simulink model "afe_rst_inv_psm_distributed_control_two_delays"  (R2026a)
settings: Solver=ode1be  StopTime=simlength  FixedStep=tc  MaxStep=Tc
values from neighbouring files (symbols this model uses):
  Amplitude_U = 1.16    [grid_fault_generator.m]
  Amplitude_V = Amplitude_U    (= 1.16)    [grid_fault_generator.m]
  Amplitude_W = Amplitude_U    (= 1.16)    [grid_fault_generator.m]
  end_time_LVRT = start_time_LVRT + error_length    [grid_fault_generator.m]
  Igrid_phase_normalization_factor = 270*sqrt(2)    [grid_emulator.m]
  omega_grid_emulator_nom = w_grid    (= 314.159265359)    [grid_emulator.m]
  omega_grid_nom = w_grid    (= 314.159265359)    [grid_emulator.m]
  t_ramp = 20e-3    (= 0.02)    [grid_fault_generator.m]
  ugrid_factor = 1    [grid_emulator.m]
  V_phase_normalization_factor = Vgrid_phase_normalization_factor    [grid_emulator.m]
  Vdc_bez = 1070    [grid_emulator.m]
  Vemu_ref_norm = Vemu_ref * sqrt(2) / V_phase_normalization_factor    [grid_emulator.m]
  vn_eta_pu = 0    [grid_emulator.m]
  vn_xi_pu = 0    [grid_emulator.m]
  vp_xi_pu = 1    [grid_emulator.m]
undefined symbols (not defined in the file or in its folder): Adrso, Aresd, Bresd, CFi, CFu, Cresd, Crso, CTRPIFF_CLIP_RELEASE, dead_time_INV, emf_fb_p, emf_fb_p_ccaller_1, emf_fb_p_ccaller_2, emf_p, emf_p_ccaller_1, emf_p_ccaller_2, fPWM_INV, g0_161Hz, g0_500Hz, g1_161Hz, g1_500Hz, i_grid_neg_eta_lim, i_grid_neg_eta_red_lim, i_grid_neg_xi_lim, i_grid_neg_xi_red_lim, i_grid_pos_eta_lim, i_grid_pos_eta_red_lim, ibez, id_lim, ieta_neg_ref_lim, ieta_pos_ref_lim, iq_lim, ixi_pos_ref_lim, Jm_norm, k_frt_ref, kg, ki_afe, ki_i, ki_id, ki_iq, ki_rc_neg_grid, ki_rc_pos_grid, ki_vs, ki_w, kp_afe, kp_i, kp_id, kp_iq, kp_rc_neg_grid, kp_rc_pos_grid, kp_vs, kp_w, kw, l1, l2, Lalpha_norm, Ld_norm, Ldrso, Lq_norm, Ls_norm, luenberger_l1 ... (+30)
libraries: fl_lib x146, nesl_utility x62, simulink x8, cstblocks_lti x7, sl_discontinuities x3, single_phase_transformer_lib x3, flexshaft_lib x1, permanent_magnet_synchronous_machine x1
(part 8 of 14)

== system afe_rst_inv_psm_distributed_control_two_delays/AFE-Modular/afe_leg_b/driver_board_b/dq_pll/pll_stageB ==
  u_grid_pos_xi : Inport
  u_grid_pos_eta : Inport  Port=2
  -2<x<2 : Saturate  UpperLimit=2  LowerLimit=-2
  Constant4 : Constant  Value=omega_grid_nom
  Product1 : Product  RndMeth=Zero
  Product2 : Product  RndMeth=Zero
  Sum3 : Sum  SaturateOnIntegerOverflow=on
  Sum4 : Sum  SaturateOnIntegerOverflow=on
  Sum5 : Sum  Inputs=++|
  Unit Delay{1..4} (4 alike) : UnitDelay  SampleTime=ts_afe
  bounder1 : MATLAB Function  TreatAsAtomicUnit=on  SystemSampleTime=ts_afe
  kp : Gain  Gain=pll_i1*ts_afe  SaturateOnIntegerOverflow=on  OutDataTypeStr=Inherit: Same as input  ParamDataTypeStr=Inherit: Same as input
  kp1 : Gain  Gain=pll_p  SaturateOnIntegerOverflow=on  OutDataTypeStr=Inherit: Same as input  ParamDataTypeStr=Inherit: Same as input
  kp2 : Gain  Gain=ts_afe  SaturateOnIntegerOverflow=on  OutDataTypeStr=Inherit: Same as input  ParamDataTypeStr=Inherit: Same as input
  gamma_grid_pll : Outport  VectorParamsAs1DForOutWhenUnconnected=off
  wires:
  Unit Delay4/1 -> Sum5/2, Sum3/2
  Sum3/1 -> -2<x<2/1
  Sum4/1 -> bounder1/1(u)
  Unit Delay1/1 -> Sum4/2
  -2<x<2/1 -> Unit Delay4/1  "i1"
  kp2/1 -> Sum4/1
  Constant4/1 -> Product2/2
  [ugrid_unorm_phase_b] -> Unit Delay2/1
  kp/1 -> Sum3/1
  Sum5/1 -> Product2/1
  u_grid_pos_eta/1 -> Unit Delay3/1
  Product2/1 -> kp2/1
  Product1/1 -> kp/1, kp1/1  "V l"
  kp1/1 -> Sum5/1
  bounder1/1(y) -> gamma_grid_pll/1, Unit Delay1/1
  Unit Delay2/1 -> Product1/2
  Unit Delay3/1 -> Product1/1

== system afe_rst_inv_psm_distributed_control_two_delays/AFE-Modular/afe_leg_b/driver_board_b/voltage-current-acquisition/is_eta_neg_ref_fieldbus ==
  is : Inport
  Unit Delay : UnitDelay  SampleTime=ts_afe
  Unit Delay1 : UnitDelay  SampleTime=ts_afe
  Zero-Order Hold : ZeroOrderHold  SampleTime=ts_afe
  is_fb : Outport
  wires:
  is/1 -> Zero-Order Hold/1
  Unit Delay/1 -> Unit Delay1/1
  Zero-Order Hold/1 -> Unit Delay/1
  Unit Delay1/1 -> is_fb/1

== system afe_rst_inv_psm_distributed_control_two_delays/AFE-Modular/afe_leg_b/driver_board_b/voltage-current-acquisition/is_eta_pos_ref_fieldbus ==
  is : Inport
  Unit Delay : UnitDelay  SampleTime=ts_afe
  Unit Delay1 : UnitDelay  SampleTime=ts_afe
  Zero-Order Hold : ZeroOrderHold  SampleTime=ts_afe
  is_fb : Outport
  wires:
  is/1 -> Zero-Order Hold/1
  Unit Delay/1 -> Unit Delay1/1
  Zero-Order Hold/1 -> Unit Delay/1
  Unit Delay1/1 -> is_fb/1

== system afe_rst_inv_psm_distributed_control_two_delays/AFE-Modular/afe_leg_b/driver_board_b/voltage-current-acquisition/is_xi_neg_ref_fieldbus ==
  is : Inport
  Unit Delay : UnitDelay  SampleTime=ts_afe
  Unit Delay1 : UnitDelay  SampleTime=ts_afe
  Zero-Order Hold : ZeroOrderHold  SampleTime=ts_afe
  is_fb : Outport
  wires:
  is/1 -> Zero-Order Hold/1
  Unit Delay/1 -> Unit Delay1/1
  Zero-Order Hold/1 -> Unit Delay/1
  Unit Delay1/1 -> is_fb/1

== system afe_rst_inv_psm_distributed_control_two_delays/AFE-Modular/afe_leg_b/driver_board_b/voltage-current-acquisition/isa_measure ==
  is : Inport
  Gain : Gain  Gain=1/Igrid_phase_normalization_factor
  Quantizer : Quantizer  QuantizationInterval=CurrentQuantization
  Unit Delay : UnitDelay  SampleTime=ts_afe
  Zero-Order Hold : ZeroOrderHold  SampleTime=ts_afe
  is_pu : Outport
  wires:
  Quantizer/1 -> Zero-Order Hold/1
  Gain/1 -> is_pu/1
  Zero-Order Hold/1 -> Unit Delay/1
  Unit Delay/1 -> Gain/1
  is/1 -> Quantizer/1

== system afe_rst_inv_psm_distributed_control_two_delays/AFE-Modular/afe_leg_b/driver_board_b/voltage-current-acquisition/isb_fieldbus ==
  is : Inport
  Unit Delay : UnitDelay  SampleTime=ts_afe
  Unit Delay1 : UnitDelay  SampleTime=ts_afe
  Zero-Order Hold : ZeroOrderHold  SampleTime=ts_afe
  is_fb : Outport
  wires:
  is/1 -> Zero-Order Hold/1
  Unit Delay/1 -> Unit Delay1/1
  Zero-Order Hold/1 -> Unit Delay/1
  Unit Delay1/1 -> is_fb/1

== system afe_rst_inv_psm_distributed_control_two_delays/AFE-Modular/afe_leg_b/driver_board_b/voltage-current-acquisition/isc_fieldbus ==
  is : Inport
  Unit Delay : UnitDelay  SampleTime=ts_afe
  Unit Delay1 : UnitDelay  SampleTime=ts_afe
  Zero-Order Hold : ZeroOrderHold  SampleTime=ts_afe
  is_fb : Outport
  wires:
  is/1 -> Zero-Order Hold/1
  Unit Delay/1 -> Unit Delay1/1
  Zero-Order Hold/1 -> Unit Delay/1
  Unit Delay1/1 -> is_fb/1

== system afe_rst_inv_psm_distributed_control_two_delays/AFE-Modular/afe_leg_b/driver_board_b/voltage-current-acquisition/ixi_ref_fieldbus ==
  is : Inport
  Unit Delay : UnitDelay  SampleTime=ts_afe
  Unit Delay1 : UnitDelay  SampleTime=ts_afe
  Zero-Order Hold : ZeroOrderHold  SampleTime=ts_afe
  is_fb : Outport
  wires:
  is/1 -> Zero-Order Hold/1
  Unit Delay/1 -> Unit Delay1/1
  Zero-Order Hold/1 -> Unit Delay/1
  Unit Delay1/1 -> is_fb/1

== system afe_rst_inv_psm_distributed_control_two_delays/AFE-Modular/afe_leg_b/driver_board_b/voltage-current-acquisition/ixi_ref_fieldbus1 ==
  is : Inport
  Unit Delay : UnitDelay  SampleTime=ts_afe
  Unit Delay1 : UnitDelay  SampleTime=ts_afe
  Zero-Order Hold : ZeroOrderHold  SampleTime=ts_afe
  is_fb : Outport
  wires:
  is/1 -> Zero-Order Hold/1
  Unit Delay/1 -> Unit Delay1/1
  Zero-Order Hold/1 -> Unit Delay/1
  Unit Delay1/1 -> is_fb/1

== system afe_rst_inv_psm_distributed_control_two_delays/AFE-Modular/afe_leg_b/driver_board_b/voltage-current-acquisition/ub_ctrl_fieldbus ==
  u_ctrl : Inport
  Unit Delay : UnitDelay  SampleTime=ts_afe
  Unit Delay1 : UnitDelay  SampleTime=ts_afe
  Zero-Order Hold : ZeroOrderHold  SampleTime=ts_afe
  u_ctrl_fb : Outport
  wires:
  u_ctrl/1 -> Zero-Order Hold/1
  Unit Delay/1 -> Unit Delay1/1
  Zero-Order Hold/1 -> Unit Delay/1
  Unit Delay1/1 -> u_ctrl_fb/1

== system afe_rst_inv_psm_distributed_control_two_delays/AFE-Modular/afe_leg_b/driver_board_b/voltage-current-acquisition/uc_ctrl_fieldbus ==
  u_ctrl : Inport
  Unit Delay : UnitDelay  SampleTime=ts_afe
  Unit Delay1 : UnitDelay  SampleTime=ts_afe
  Zero-Order Hold : ZeroOrderHold  SampleTime=ts_afe
  u_ctrl_fb : Outport
  wires:
  u_ctrl/1 -> Zero-Order Hold/1
  Unit Delay/1 -> Unit Delay1/1
  Zero-Order Hold/1 -> Unit Delay/1
  Unit Delay1/1 -> u_ctrl_fb/1

== system afe_rst_inv_psm_distributed_control_two_delays/AFE-Modular/afe_leg_b/driver_board_b/voltage-current-acquisition/uga_measure ==
  ug : Inport
  Gain : Gain  Gain=1/V_phase_normalization_factor
  Quantizer : Quantizer  QuantizationInterval=CurrentQuantization
  Unit Delay : UnitDelay  SampleTime=ts_afe
  Zero-Order Hold : ZeroOrderHold  SampleTime=ts_afe
  ug_pu : Outport
  wires:
  ug/1 -> Quantizer/1
  Unit Delay/1 -> Gain/1
  Zero-Order Hold/1 -> Unit Delay/1
  Gain/1 -> ug_pu/1
  Quantizer/1 -> Zero-Order Hold/1

== system afe_rst_inv_psm_distributed_control_two_delays/AFE-Modular/afe_leg_b/driver_board_b/voltage-current-acquisition/ugb_fieldbus ==
  ug : Inport
  Unit Delay : UnitDelay  SampleTime=ts_afe
  Unit Delay1 : UnitDelay  SampleTime=ts_afe
  Zero-Order Hold : ZeroOrderHold  SampleTime=ts_afe
  ug_fb : Outport
  wires:
  ug/1 -> Zero-Order Hold/1
  Unit Delay/1 -> Unit Delay1/1
  Zero-Order Hold/1 -> Unit Delay/1
  Unit Delay1/1 -> ug_fb/1

== system afe_rst_inv_psm_distributed_control_two_delays/AFE-Modular/afe_leg_b/driver_board_b/voltage-current-acquisition/ugc_fieldbus ==
  ug : Inport
  Unit Delay : UnitDelay  SampleTime=ts_afe
  Unit Delay1 : UnitDelay  SampleTime=ts_afe
  Zero-Order Hold : ZeroOrderHold  SampleTime=ts_afe
  ug_fb : Outport
  wires:
  ug/1 -> Zero-Order Hold/1
  Unit Delay/1 -> Unit Delay1/1
  Zero-Order Hold/1 -> Unit Delay/1
  Unit Delay1/1 -> ug_fb/1

== system afe_rst_inv_psm_distributed_control_two_delays/AFE-Modular/afe_leg_b/modulator/sv_pwm/modulator ==
  u : Inport
  v : Inport  Port=2
  w : Inport  Port=3
  Bus Creator : BusCreator  Inputs=6
  PWM generator 1 : Subsystem  mask{f=fPWM_INV, ph=0, m_up=0.98, m_low=0.02, dead_time=dead_time_INV, vg_firing=15, polarity=1}
      mask prompts: f "Frequency"; ph "Phase"; m_up "Max Input Modulation Value"; m_low "Min Input Modulation Value"; dead_time "Dead Time"; vg_firing "Gate Voltage"
  PWM generator 2 : Subsystem  mask{f=fPWM_INV, ph=0, m_up=0.98, m_low=0.02, dead_time=dead_time_INV, vg_firing=15, polarity=1}
      mask prompts: f "Frequency"; ph "Phase"; m_up "Max Input Modulation Value"; m_low "Min Input Modulation Value"; dead_time "Dead Time"; vg_firing "Gate Voltage"
  PWM generator 3 : Subsystem  mask{f=fPWM_INV, ph=0, m_up=0.98, m_low=0.02, dead_time=dead_time_INV, vg_firing=15, polarity=1}
      mask prompts: f "Frequency"; ph "Phase"; m_up "Max Input Modulation Value"; m_low "Min Input Modulation Value"; dead_time "Dead Time"; vg_firing "Gate Voltage"
  firing_gates : Outport
  wires:
  PWM generator 1/1(m1) -> Bus Creator/1  "pwm_u_top"
  PWM generator 3/2(m2) -> Bus Creator/6  "pwm_w_bottom"
  PWM generator 2/2(m2) -> Bus Creator/4  "pwm_v_bottom"
  PWM generator 3/1(m1) -> Bus Creator/5  "pwm_w_top"
  PWM generator 2/1(m1) -> Bus Creator/3  "pwm_v_top"
  Bus Creator/1 -> firing_gates/1
  PWM generator 1/2(m2) -> Bus Creator/2  "pwm_u_bottom"
  v/1 -> PWM generator 2/1(m_index)
  w/1 -> PWM generator 3/1(m_index)
  u/1 -> PWM generator 1/1(m_index)

== system afe_rst_inv_psm_distributed_control_two_delays/AFE-Modular/afe_leg_c/driver_board_c/current_ctrl/phase_current_control ==
  In1 : Inport
  is_abc : Inport  Port=2
  Bus Creator1 : BusCreator  Inputs=2
  Bus Creator2 : BusCreator  Inputs=3
  Bus Selector1 : BusSelector  OutputSignals=usa_ctrl,usb_ctrl,usc_ctrl
  MATLAB Function : MATLAB Function  TreatAsAtomicUnit=on
  Selector : Selector  InputPortWidth=3  IndexOptions=Index vector (dialog)  Indices=3  OutputSizes=1
  Unit Delay2 : UnitDelay  SampleTime=ts_afe
  Unit Delay3 : UnitDelay  SampleTime=ts_afe
  isc_ref/isc : Scope  NumInputPorts=2
      settings: SampleTime=ts_afe  ActiveDisplayYMinimum=-6.6016  ActiveDisplayYMaximum=2.92896
  phase-current-control-dbc : Subsystem
  us_alphabeta_ctrl : Outport  VectorParamsAs1DForOutWhenUnconnected=off
  tag scope: usc_ctrl_dbc=global
  wires:
  Bus Creator1/1 -> us_alphabeta_ctrl/1
  Unit Delay2/1 -> Bus Creator1/1  "us_alpha_ctrl"
  Bus Selector1/1 -> MATLAB Function/1(a)  "<usa_ctrl>"
  MATLAB Function/2(beta) -> Unit Delay3/1
  Bus Selector1/2 -> MATLAB Function/2(b)  "<usb_ctrl>"
  Unit Delay3/1 -> Bus Creator1/2  "us_beta_ctrl"
  MATLAB Function/1(alpha) -> Unit Delay2/1
  Bus Selector1/3 -> MATLAB Function/3(c)  "<usc_ctrl>"
  is_abc/1 -> isc_ref/isc/2, phase-current-control-dbc/2(is_abc)  "isc"
  In1/1 -> Selector/1
  phase-current-control-dbc/1(Out1) -> Bus Creator2/3, [usc_ctrl_dbc]  "usc_ctrl"
  [usb_ctrl_dbb_fb_dbc] -> Bus Creator2/2  "usb_ctrl"
  [usa_ctrl_dba_fb_dbc] -> Bus Creator2/1  "usa_ctrl"
  Bus Creator2/1 -> Bus Selector1/1  "us_abc_ctrl"
  Selector/1 -> isc_ref/isc/1, phase-current-control-dbc/1(In1)  "isc_ref"

== system afe_rst_inv_psm_distributed_control_two_delays/AFE-Modular/afe_leg_c/driver_board_c/current_ctrl/xieta2abc ==
  pos_xi : Inport
  pos_eta : Inport  Port=2
  neg_xi : Inport  Port=3
  neg_eta : Inport  Port=4
  gamma : Inport  Port=5
  MATLAB Function2 : MATLAB Function  TreatAsAtomicUnit=on
  Mux : Mux  Inputs=3
  Negative Sequence : MATLAB Function  TreatAsAtomicUnit=on
  Positive Sequence : MATLAB Function  TreatAsAtomicUnit=on
  Sum : Sum  Inputs=|++
  Sum1 : Sum  Inputs=|++
  i_abc_reference : Outport
  wires:
  Mux/1 -> i_abc_reference/1  "i_abc_reference"
  pos_eta/1 -> Positive Sequence/2(eta)
  pos_xi/1 -> Positive Sequence/1(xi)
  neg_xi/1 -> Negative Sequence/1(xi)
  Sum1/1 -> MATLAB Function2/2(beta)
  MATLAB Function2/2(b) -> Mux/2  "i_b"
  Negative Sequence/2(beta) -> Sum1/2
  Positive Sequence/1(alpha) -> Sum/1
  Negative Sequence/1(alpha) -> Sum/2
  MATLAB Function2/3(c) -> Mux/3  "i_c"
  gamma/1 -> Positive Sequence/3(gamma), Negative Sequence/3(gamma)
  Sum/1 -> MATLAB Function2/1(alpha)
  Positive Sequence/2(beta) -> Sum1/1
  MATLAB Function2/1(a) -> Mux/1  "i_a"
  neg_eta/1 -> Negative Sequence/2(eta)

== system afe_rst_inv_psm_distributed_control_two_delays/AFE-Modular/afe_leg_c/driver_board_c/dq_pll/pll_stageA ==
  gamma_grid : Inport
  Math Function : Math  Operator=magnitude^2  SignedPower=on
  Math Function1 : Math  Operator=magnitude^2  SignedPower=on
  Reciprocal Sqrt : Sqrt  Operator=rSqrt
  Saturation : Saturate  UpperLimit=inf  LowerLimit=0.02
  Sum : Sum  Inputs=|++
  mormalization_and_transformation : Subsystem
  sequences : Subsystem
  u_grid_pos_xi : Outport  VectorParamsAs1DForOutWhenUnconnected=off
  u_grid_pos_eta : Outport  Port=2  VectorParamsAs1DForOutWhenUnconnected=off
  tag scope: ugrid_unorm_phase_c=global
  wires:
  mormalization_and_transformation/1(ug_alpha) -> Math Function/1, sequences/1(u_grid_alpha)
  mormalization_and_transformation/2(ug_beta) -> Math Function1/1, sequences/2(u_grid_beta)
  Math Function/1 -> Sum/1
  Math Function1/1 -> Sum/2
  Sum/1 -> Saturation/1
  Reciprocal Sqrt/1 -> [ugrid_unorm_phase_c]
  Saturation/1 -> Reciprocal Sqrt/1
  gamma_grid/1 -> sequences/3(gamma_grid)
  sequences/1(u_grid_pos_xi) -> u_grid_pos_xi/1
  sequences/2(u_grid_pos_eta) -> u_grid_pos_eta/1
  [ugb_pu_dbb_fb_dbc] -> mormalization_and_transformation/2(ug_b)
  [uga_pu_dba_fb_dbc] -> mormalization_and_transformation/1(ug_a)
  [ugc_pu_dbc] -> mormalization_and_transformation/3(ug_c)

== system afe_rst_inv_psm_distributed_control_two_delays/AFE-Modular/afe_leg_c/driver_board_c/dq_pll/pll_stageB ==
  u_grid_pos_xi : Inport
  u_grid_pos_eta : Inport  Port=2
  -2<x<2 : Saturate  UpperLimit=2  LowerLimit=-2
  Constant4 : Constant  Value=omega_grid_nom
  Product1 : Product  RndMeth=Zero
  Product2 : Product  RndMeth=Zero
  Sum3 : Sum  SaturateOnIntegerOverflow=on
  Sum4 : Sum  SaturateOnIntegerOverflow=on
  Sum5 : Sum  Inputs=++|
  Unit Delay{1..4} (4 alike) : UnitDelay  SampleTime=ts_afe
  bounder1 : MATLAB Function  TreatAsAtomicUnit=on  SystemSampleTime=ts_afe
  kp : Gain  Gain=pll_i1*ts_afe  SaturateOnIntegerOverflow=on  OutDataTypeStr=Inherit: Same as input  ParamDataTypeStr=Inherit: Same as input
  kp1 : Gain  Gain=pll_p  SaturateOnIntegerOverflow=on  OutDataTypeStr=Inherit: Same as input  ParamDataTypeStr=Inherit: Same as input
  kp2 : Gain  Gain=ts_afe  SaturateOnIntegerOverflow=on  OutDataTypeStr=Inherit: Same as input  ParamDataTypeStr=Inherit: Same as input
  gamma_grid_pll : Outport  VectorParamsAs1DForOutWhenUnconnected=off
  wires:
  Unit Delay4/1 -> Sum3/2, Sum5/2
  Sum3/1 -> -2<x<2/1
  Sum4/1 -> bounder1/1(u)
  Unit Delay1/1 -> Sum4/2
  -2<x<2/1 -> Unit Delay4/1  "i1"
  kp2/1 -> Sum4/1
  Constant4/1 -> Product2/2
  [ugrid_unorm_phase_c] -> Unit Delay2/1
  kp/1 -> Sum3/1
  Sum5/1 -> Product2/1
  u_grid_pos_eta/1 -> Unit Delay3/1
  Product2/1 -> kp2/1
  Product1/1 -> kp/1, kp1/1  "V l"
  kp1/1 -> Sum5/1
  bounder1/1(y) -> gamma_grid_pll/1, Unit Delay1/1
  Unit Delay2/1 -> Product1/2
  Unit Delay3/1 -> Product1/1

== system afe_rst_inv_psm_distributed_control_two_delays/AFE-Modular/afe_leg_c/driver_board_c/voltage-current-acquisition/is_eta_neg_ref_fieldbus ==
  is : Inport
  Unit Delay : UnitDelay  SampleTime=ts_afe
  Unit Delay1 : UnitDelay  SampleTime=ts_afe
  Zero-Order Hold : ZeroOrderHold  SampleTime=ts_afe
  is_fb : Outport
  wires:
  is/1 -> Zero-Order Hold/1
  Unit Delay/1 -> Unit Delay1/1
  Zero-Order Hold/1 -> Unit Delay/1
  Unit Delay1/1 -> is_fb/1

== system afe_rst_inv_psm_distributed_control_two_delays/AFE-Modular/afe_leg_c/driver_board_c/voltage-current-acquisition/is_eta_pos_ref_fieldbus ==
  is : Inport
  Unit Delay : UnitDelay  SampleTime=ts_afe
  Unit Delay1 : UnitDelay  SampleTime=ts_afe
  Zero-Order Hold : ZeroOrderHold  SampleTime=ts_afe
  is_fb : Outport
  wires:
  is/1 -> Zero-Order Hold/1
  Unit Delay/1 -> Unit Delay1/1
  Zero-Order Hold/1 -> Unit Delay/1
  Unit Delay1/1 -> is_fb/1

== system afe_rst_inv_psm_distributed_control_two_delays/AFE-Modular/afe_leg_c/driver_board_c/voltage-current-acquisition/is_xi_neg_ref_fieldbus ==
  is : Inport
  Unit Delay : UnitDelay  SampleTime=ts_afe
  Unit Delay1 : UnitDelay  SampleTime=ts_afe
  Zero-Order Hold : ZeroOrderHold  SampleTime=ts_afe
  is_fb : Outport
  wires:
  is/1 -> Zero-Order Hold/1
  Unit Delay/1 -> Unit Delay1/1
  Zero-Order Hold/1 -> Unit Delay/1
  Unit Delay1/1 -> is_fb/1

== system afe_rst_inv_psm_distributed_control_two_delays/AFE-Modular/afe_leg_c/driver_board_c/voltage-current-acquisition/isb_fieldbus ==
  is : Inport
  Unit Delay : UnitDelay  SampleTime=ts_afe
  Unit Delay1 : UnitDelay  SampleTime=ts_afe
  Zero-Order Hold : ZeroOrderHold  SampleTime=ts_afe
  is_fb : Outport
  wires:
  is/1 -> Zero-Order Hold/1
  Unit Delay/1 -> Unit Delay1/1
  Zero-Order Hold/1 -> Unit Delay/1
  Unit Delay1/1 -> is_fb/1

== system afe_rst_inv_psm_distributed_control_two_delays/AFE-Modular/afe_leg_c/driver_board_c/voltage-current-acquisition/isc_fieldbus ==
  is : Inport
  Unit Delay : UnitDelay  SampleTime=ts_afe
  Unit Delay1 : UnitDelay  SampleTime=ts_afe
  Zero-Order Hold : ZeroOrderHold  SampleTime=ts_afe
  is_fb : Outport
  wires:
  is/1 -> Zero-Order Hold/1
  Unit Delay/1 -> Unit Delay1/1
  Zero-Order Hold/1 -> Unit Delay/1
  Unit Delay1/1 -> is_fb/1

== system afe_rst_inv_psm_distributed_control_two_delays/AFE-Modular/afe_leg_c/driver_board_c/voltage-current-acquisition/isc_measure_and_normalization ==
  is : Inport
  Gain : Gain  Gain=1/Igrid_phase_normalization_factor
  Quantizer : Quantizer  QuantizationInterval=CurrentQuantization
  Unit Delay : UnitDelay  SampleTime=ts_afe
  Zero-Order Hold : ZeroOrderHold  SampleTime=ts_afe
  is_pu : Outport
  wires:
  Quantizer/1 -> Zero-Order Hold/1
  Gain/1 -> is_pu/1
  Zero-Order Hold/1 -> Unit Delay/1
  Unit Delay/1 -> Gain/1
  is/1 -> Quantizer/1

== system afe_rst_inv_psm_distributed_control_two_delays/AFE-Modular/afe_leg_c/driver_board_c/voltage-current-acquisition/ixi_ref_fieldbus ==
  is : Inport
  Unit Delay : UnitDelay  SampleTime=ts_afe
  Unit Delay1 : UnitDelay  SampleTime=ts_afe
  Zero-Order Hold : ZeroOrderHold  SampleTime=ts_afe
  is_fb : Outport
  wires:
  is/1 -> Zero-Order Hold/1
  Unit Delay/1 -> Unit Delay1/1
  Zero-Order Hold/1 -> Unit Delay/1
  Unit Delay1/1 -> is_fb/1

== system afe_rst_inv_psm_distributed_control_two_delays/AFE-Modular/afe_leg_c/driver_board_c/voltage-current-acquisition/ixi_ref_fieldbus1 ==
  is : Inport
  Unit Delay : UnitDelay  SampleTime=ts_afe
  Unit Delay1 : UnitDelay  SampleTime=ts_afe
  Zero-Order Hold : ZeroOrderHold  SampleTime=ts_afe
  is_fb : Outport
  wires:
  is/1 -> Zero-Order Hold/1
  Unit Delay/1 -> Unit Delay1/1
  Zero-Order Hold/1 -> Unit Delay/1
  Unit Delay1/1 -> is_fb/1

== system afe_rst_inv_psm_distributed_control_two_delays/AFE-Modular/afe_leg_c/driver_board_c/voltage-current-acquisition/ub_ctrl_fieldbus ==
  u_ctrl : Inport
  Unit Delay : UnitDelay  SampleTime=ts_afe
  Unit Delay1 : UnitDelay  SampleTime=ts_afe
  Zero-Order Hold : ZeroOrderHold  SampleTime=ts_afe
  u_ctrl_fb : Outport
  wires:
  u_ctrl/1 -> Zero-Order Hold/1
  Unit Delay/1 -> Unit Delay1/1
  Zero-Order Hold/1 -> Unit Delay/1
  Unit Delay1/1 -> u_ctrl_fb/1

== system afe_rst_inv_psm_distributed_control_two_delays/AFE-Modular/afe_leg_c/driver_board_c/voltage-current-acquisition/uc_ctrl_fieldbus ==
  u_ctrl : Inport
  Unit Delay : UnitDelay  SampleTime=ts_afe
  Unit Delay1 : UnitDelay  SampleTime=ts_afe
  Zero-Order Hold : ZeroOrderHold  SampleTime=ts_afe
  u_ctrl_fb : Outport
  wires:
  u_ctrl/1 -> Zero-Order Hold/1
  Unit Delay/1 -> Unit Delay1/1
  Zero-Order Hold/1 -> Unit Delay/1
  Unit Delay1/1 -> u_ctrl_fb/1

== system afe_rst_inv_psm_distributed_control_two_delays/AFE-Modular/afe_leg_c/driver_board_c/voltage-current-acquisition/uga_fieldbus ==
  ug : Inport
  Unit Delay : UnitDelay  SampleTime=ts_afe
  Unit Delay1 : UnitDelay  SampleTime=ts_afe
  Zero-Order Hold : ZeroOrderHold  SampleTime=ts_afe
  ug_fb : Outport
  wires:
  ug/1 -> Zero-Order Hold/1
  Zero-Order Hold/1 -> Unit Delay/1
  Unit Delay/1 -> Unit Delay1/1
  Unit Delay1/1 -> ug_fb/1

== system afe_rst_inv_psm_distributed_control_two_delays/AFE-Modular/afe_leg_c/driver_board_c/voltage-current-acquisition/ugb_fieldbus ==
  ug : Inport
  Unit Delay : UnitDelay  SampleTime=ts_afe
  Unit Delay1 : UnitDelay  SampleTime=ts_afe
  Zero-Order Hold : ZeroOrderHold  SampleTime=ts_afe
  ug_fb : Outport
  wires:
  ug/1 -> Zero-Order Hold/1
  Unit Delay/1 -> Unit Delay1/1
  Zero-Order Hold/1 -> Unit Delay/1
  Unit Delay1/1 -> ug_fb/1

== system afe_rst_inv_psm_distributed_control_two_delays/AFE-Modular/afe_leg_c/driver_board_c/voltage-current-acquisition/ugc_measure_and_normalization ==
  ug : Inport
  Gain : Gain  Gain=1/V_phase_normalization_factor
  Quantizer : Quantizer  QuantizationInterval=CurrentQuantization
  Unit Delay : UnitDelay  SampleTime=ts_afe
  Zero-Order Hold : ZeroOrderHold  SampleTime=ts_afe
  ug_pu : Outport
  wires:
  ug/1 -> Quantizer/1
  Unit Delay/1 -> Gain/1
  Zero-Order Hold/1 -> Unit Delay/1
  Gain/1 -> ug_pu/1
  Quantizer/1 -> Zero-Order Hold/1

== system afe_rst_inv_psm_distributed_control_two_delays/AFE-Modular/afe_leg_c/modulator/sv_pwm/modulator ==
  u : Inport
  v : Inport  Port=2
  w : Inport  Port=3
  Bus Creator : BusCreator  Inputs=6
  PWM generator 1 : Subsystem  mask{f=fPWM_INV, ph=0, m_up=0.98, m_low=0.02, dead_time=dead_time_INV, vg_firing=15, polarity=1}
      mask prompts: f "Frequency"; ph "Phase"; m_up "Max Input Modulation Value"; m_low "Min Input Modulation Value"; dead_time "Dead Time"; vg_firing "Gate Voltage"
  PWM generator 2 : Subsystem  mask{f=fPWM_INV, ph=0, m_up=0.98, m_low=0.02, dead_time=dead_time_INV, vg_firing=15, polarity=1}
      mask prompts: f "Frequency"; ph "Phase"; m_up "Max Input Modulation Value"; m_low "Min Input Modulation Value"; dead_time "Dead Time"; vg_firing "Gate Voltage"
  PWM generator 3 : Subsystem  mask{f=fPWM_INV, ph=0, m_up=0.98, m_low=0.02, dead_time=dead_time_INV, vg_firing=15, polarity=1}
      mask prompts: f "Frequency"; ph "Phase"; m_up "Max Input Modulation Value"; m_low "Min Input Modulation Value"; dead_time "Dead Time"; vg_firing "Gate Voltage"
  firing_gates : Outport
  wires:
  u/1 -> PWM generator 1/1(m_index)
  w/1 -> PWM generator 3/1(m_index)
  v/1 -> PWM generator 2/1(m_index)
  PWM generator 1/2(m2) -> Bus Creator/2  "pwm_u_bottom"
  Bus Creator/1 -> firing_gates/1
  PWM generator 2/1(m1) -> Bus Creator/3  "pwm_v_top"
  PWM generator 3/1(m1) -> Bus Creator/5  "pwm_w_top"
  PWM generator 2/2(m2) -> Bus Creator/4  "pwm_v_bottom"
  PWM generator 3/2(m2) -> Bus Creator/6  "pwm_w_bottom"
  PWM generator 1/1(m1) -> Bus Creator/1  "pwm_u_top"

== system afe_rst_inv_psm_distributed_control_two_delays/INV-Modular/inv_leg_u/driver_board_u/motor_vector_control/bemf_observer ==
  ialpha_pu : Inport
  ibeta_pu : Inport  Port=2
  ualpha_pu : Inport  Port=3
  ubeta_pu : Inport  Port=4
  Unit Delay : UnitDelay  SampleTime=ts_inv
  Unit Delay1 : UnitDelay  SampleTime=ts_inv
  bemf_observer_ccaller : Subsystem  Commented=on
  bemf_observer_simulink : Subsystem
  bemf_observer_with_load_estimator_ccaller : Subsystem  Commented=on
  tag scope: motor_omega_hat_pu_dbu=global, motor_theta_hat_dbu=global
  wires:
  ialpha_pu/1 -> bemf_observer_simulink/1(ialpha_pu)
  ibeta_pu/1 -> bemf_observer_simulink/2(ibeta_pu)
  ualpha_pu/1 -> bemf_observer_simulink/3(ualpha_pu)
  ubeta_pu/1 -> bemf_observer_simulink/4(ubeta_pu)
  bemf_observer_simulink/2(theta_hat) -> Unit Delay1/1  "theta_hat"
  bemf_observer_simulink/1(omega_pu_hat) -> Unit Delay/1  "omega_hat_pu"
  Unit Delay/1 -> [motor_omega_hat_pu_dbu]
  Unit Delay1/1 -> [motor_theta_hat_dbu]

== system afe_rst_inv_psm_distributed_control_two_delays/INV-Modular/inv_leg_u/driver_board_u/motor_vector_control/current_ctrl ==
  iq_ref : Inport
  MTPA : Subsystem
      mask Display: disp('MTPA')
  Sqrt : Sqrt
  Square : Math  Operator=square
  Square1 : Math  Operator=square
  Sum : Sum  Inputs=|++
  To Workspace7 : ToWorkspace  VariableName=u_mot_pu_sim  SampleTime=ts_inv
      settings: MaxDataPoints=Ns_inv
  dq_pi_with_vector_antiwindup : Subsystem
  id_ref : Subsystem
      settings: PortSchema="{\"entries\":[{\"content\":{\"sides\":[{\"content\":{},\"type\":\"ConnectorPlacement.EquallySpacedRectSide\",\"uuid\":\"42af5d69-f0eb-42c6-9e03-28c1d0757323\"},{\"content\":{\"connectorIds\":[\"Out1\"],\"side\":\"RIGHT\"},\"type\":\"ConnectorPlacement.EquallySpacedRectSide\",\"uuid\":\"dd68a9f9-d15f-4e57-9d9e-130889a7b90c\"},{\"content\":{\"connectorIds\":[\"In1\"],\"side\":\"TOP\"},\"type\":\"ConnectorPlacement.EquallySpacedRectSide\",\"uuid\":\"68c797a2-8439-4b8d-8368-b7485adf0676\"}]},\"type\":\"ConnectorPlacement.EquallySpacedConnector\",\"uuid\":\"693c5f1c-0580-4626-8f13-b27865dfb3ac\"}],\"packageUris\":[\"http://schema.mathworks.com/mf0/Connector/R2020b\"],\"version\":\"1.0\"}"
  idref/id : Scope  NumInputPorts=2
      settings: SampleTime=tc  ActiveDisplayYMinimum=-0.16984  ActiveDisplayYMaximum=0.0865
  iqref/iq : Scope  NumInputPorts=2
      settings: SampleTime=tc  ActiveDisplayYMinimum=-0.66775  ActiveDisplayYMaximum=0.07588  DataLoggingVariableName=ScopeData2
  ud : Outport
  uq : Outport  Port=2
  wires:
  [motor_iq_pu_dbu] -> iqref/iq/2, dq_pi_with_vector_antiwindup/4(iq)  "iq"
  [motor_id_pu_dbu] -> idref/id/2, dq_pi_with_vector_antiwindup/2(id)  "id"
  MTPA/1(Id_ref_mtpa) -> id_ref/1(id_mtpa)  "id_ref"
  dq_pi_with_vector_antiwindup/1(ctrl_d_u) -> Square1/1, ud/1
  dq_pi_with_vector_antiwindup/2(ctrl_q_u) -> Square/1, uq/1
  Square/1 -> Sum/1
  Sum/1 -> Sqrt/1
  Square1/1 -> Sum/2
  Sqrt/1 -> To Workspace7/1
  id_ref/1(id_ref) -> dq_pi_with_vector_antiwindup/1(id_ref), idref/id/1
  iq_ref/1 -> iqref/iq/1, dq_pi_with_vector_antiwindup/3(iq_ref)  "iq_ref"
  [motor_iq_pu_dbu] -> MTPA/1(iq)  "iq"

== system afe_rst_inv_psm_distributed_control_two_delays/INV-Modular/inv_leg_u/driver_board_u/motor_vector_control/current_transformation ==
  u : Inport
  v : Inport  Port=2
  w : Inport  Port=3
  gamma : Inport  Port=4
  alphabeta2dq : MATLAB Function  TreatAsAtomicUnit=on  SystemSampleTime=ts_inv
  uvw2alphabeta : MATLAB Function  TreatAsAtomicUnit=on  SystemSampleTime=ts_inv
  tag scope: motor_ialpha_pu_dbu=global, motor_ibeta_pu_dbu=global, motor_id_pu_dbu=global, motor_iq_pu_dbu=global
  wires:
  w/1 -> uvw2alphabeta/3(w)
  alphabeta2dq/2(q) -> [motor_iq_pu_dbu]  "iq_pu"
  alphabeta2dq/1(d) -> [motor_id_pu_dbu]  "id_pu"
  v/1 -> uvw2alphabeta/2(v)
  uvw2alphabeta/2(beta) -> [motor_ibeta_pu_dbu], alphabeta2dq/2(beta)  "ibeta_pu"
  uvw2alphabeta/1(alpha) -> [motor_ialpha_pu_dbu], alphabeta2dq/1(alpha)  "ialpha_pu"
  u/1 -> uvw2alphabeta/1(u)
  gamma/1 -> alphabeta2dq/3(gamma)

== system afe_rst_inv_psm_distributed_control_two_delays/INV-Modular/inv_leg_u/driver_board_u/torque_curve/omega_hat_flt ==
  omega_hat : Inport
  Gain3 : Gain  Gain=omega_flt_g1
  Gain6 : Gain  Gain=omega_flt_g0
  Sum : Sum  Inputs=|++
  Unit Delay1 : UnitDelay  SampleTime=ts_inv
  omega_hat_flt : Outport  VectorParamsAs1DForOutWhenUnconnected=off
  wires:
  Sum/1 -> omega_hat_flt/1, Unit Delay1/1
  Gain3/1 -> Sum/2
  Unit Delay1/1 -> Gain3/1
  omega_hat/1 -> Gain6/1
  Gain6/1 -> Sum/1

== system afe_rst_inv_psm_distributed_control_two_delays/INV-Modular/inv_leg_u/driver_board_u/voltage-current-acquisition/isu_measure ==
  is : Inport
  Gain : Gain  Gain=1/ibez
  Quantizer : Quantizer  QuantizationInterval=CurrentQuantization
  Unit Delay : UnitDelay  SampleTime=ts_afe
  Zero-Order Hold : ZeroOrderHold  SampleTime=ts_afe
  is_pu : Outport
  wires:
  is/1 -> Quantizer/1
  Unit Delay/1 -> Gain/1
  Zero-Order Hold/1 -> Unit Delay/1
  Gain/1 -> is_pu/1
  Quantizer/1 -> Zero-Order Hold/1

== system afe_rst_inv_psm_distributed_control_two_delays/INV-Modular/inv_leg_u/driver_board_u/voltage-current-acquisition/isv_fieldbus ==
  is : Inport
  Unit Delay : UnitDelay  SampleTime=ts_inv
  Unit Delay1 : UnitDelay  SampleTime=ts_inv
  Zero-Order Hold : ZeroOrderHold  SampleTime=ts_inv
  is_fb : Outport
  wires:
  Zero-Order Hold/1 -> Unit Delay/1
  is/1 -> Zero-Order Hold/1
  Unit Delay/1 -> Unit Delay1/1
  Unit Delay1/1 -> is_fb/1

== system afe_rst_inv_psm_distributed_control_two_delays/INV-Modular/inv_leg_u/driver_board_u/voltage-current-acquisition/isw_fieldbus ==
  is : Inport
  Unit Delay : UnitDelay  SampleTime=ts_inv
  Unit Delay1 : UnitDelay  SampleTime=ts_inv
  Zero-Order Hold : ZeroOrderHold  SampleTime=ts_inv
  is_fb : Outport
  wires:
  Zero-Order Hold/1 -> Unit Delay/1
  is/1 -> Zero-Order Hold/1
  Unit Delay/1 -> Unit Delay1/1
  Unit Delay1/1 -> is_fb/1

== system afe_rst_inv_psm_distributed_control_two_delays/INV-Modular/inv_leg_u/driver_board_u/voltage-current-acquisition/motor_phase_fieldbus ==
  motor_phase : Inport
  Unit Delay : UnitDelay  SampleTime=ts_inv
  Unit Delay1 : UnitDelay  SampleTime=ts_inv
  Zero-Order Hold : ZeroOrderHold  SampleTime=ts_inv
  motor_phase_fb : Outport
  wires:
  Zero-Order Hold/1 -> Unit Delay/1
  motor_phase/1 -> Zero-Order Hold/1
  Unit Delay/1 -> Unit Delay1/1
  Unit Delay1/1 -> motor_phase_fb/1

== system afe_rst_inv_psm_distributed_control_two_delays/INV-Modular/inv_leg_u/driver_board_u/voltage-current-acquisition/usu_measure ==
  us : Inport
  Gain : Gain  Gain=1/ubez
  Quantizer : Quantizer  QuantizationInterval=CurrentQuantization
  Unit Delay : UnitDelay  SampleTime=ts_inv
  Zero-Order Hold : ZeroOrderHold  SampleTime=ts_inv
  us_pu : Outport
  wires:
  Quantizer/1 -> Zero-Order Hold/1
  Gain/1 -> us_pu/1
  Zero-Order Hold/1 -> Unit Delay/1
  Unit Delay/1 -> Gain/1
  us/1 -> Quantizer/1

== system afe_rst_inv_psm_distributed_control_two_delays/INV-Modular/inv_leg_u/driver_board_u/voltage-current-acquisition/usv_ctrl_fieldbus ==
  u_ctrl : Inport
  Unit Delay : UnitDelay  SampleTime=ts_inv
  Unit Delay1 : UnitDelay  SampleTime=ts_inv
  Zero-Order Hold : ZeroOrderHold  SampleTime=ts_inv
  u_ctrl_fb : Outport
  wires:
  Zero-Order Hold/1 -> Unit Delay/1
  u_ctrl/1 -> Zero-Order Hold/1
  Unit Delay/1 -> Unit Delay1/1
  Unit Delay1/1 -> u_ctrl_fb/1

== system afe_rst_inv_psm_distributed_control_two_delays/INV-Modular/inv_leg_u/driver_board_u/voltage-current-acquisition/usv_fieldbus ==
  us : Inport
  Unit Delay : UnitDelay  SampleTime=ts_inv
  Unit Delay1 : UnitDelay  SampleTime=ts_inv
  Zero-Order Hold : ZeroOrderHold  SampleTime=ts_inv
  us_fb : Outport
  wires:
  Zero-Order Hold/1 -> Unit Delay/1
  us/1 -> Zero-Order Hold/1
  Unit Delay/1 -> Unit Delay1/1
  Unit Delay1/1 -> us_fb/1

== system afe_rst_inv_psm_distributed_control_two_delays/INV-Modular/inv_leg_u/driver_board_u/voltage-current-acquisition/usw_ctrl_fieldbus ==
  u_ctrl : Inport
  Unit Delay : UnitDelay  SampleTime=ts_inv
  Unit Delay1 : UnitDelay  SampleTime=ts_inv
  Zero-Order Hold : ZeroOrderHold  SampleTime=ts_inv
  u_ctrl_fb : Outport
  wires:
  Zero-Order Hold/1 -> Unit Delay/1
  u_ctrl/1 -> Zero-Order Hold/1
  Unit Delay/1 -> Unit Delay1/1
  Unit Delay1/1 -> u_ctrl_fb/1

== system afe_rst_inv_psm_distributed_control_two_delays/INV-Modular/inv_leg_u/driver_board_u/voltage-current-acquisition/usw_fieldbus ==
  us : Inport
  Unit Delay : UnitDelay  SampleTime=ts_inv
  Unit Delay1 : UnitDelay  SampleTime=ts_inv
  Zero-Order Hold1 : ZeroOrderHold  SampleTime=ts_inv
  us_fb : Outport
  wires:
  Zero-Order Hold1/1 -> Unit Delay/1
  us/1 -> Zero-Order Hold1/1
  Unit Delay/1 -> Unit Delay1/1
  Unit Delay1/1 -> us_fb/1

== system afe_rst_inv_psm_distributed_control_two_delays/INV-Modular/inv_leg_u/modulator/sv_pwm/modulator ==
  u : Inport
  Bus Creator : BusCreator  Inputs=2
  PWM generator : Subsystem  mask{f=fPWM_INV, ph=0, m_up=0.98, m_low=0.02, dead_time=dead_time_INV, vg_firing=15, polarity=1}
      mask prompts: f "Frequency"; ph "Phase"; m_up "Max Input Modulation Value"; m_low "Min Input Modulation Value"; dead_time "Dead Time"; vg_firing "Gate Voltage"
  firing_gates : Outport
  wires:
  PWM generator/1(m1) -> Bus Creator/1  "pwm_u_top"
  Bus Creator/1 -> firing_gates/1
  PWM generator/2(m2) -> Bus Creator/2  "pwm_u_bottom"
  u/1 -> PWM generator/1(m_index)

== system afe_rst_inv_psm_distributed_control_two_delays/INV-Modular/inv_leg_v/driver_board_v/motor_vector_control/bemf_observer ==
  ialpha_pu : Inport
  ibeta_pu : Inport  Port=2
  ualpha_pu : Inport  Port=3
  ubeta_pu : Inport  Port=4
  Unit Delay : UnitDelay  SampleTime=ts_inv
  Unit Delay1 : UnitDelay  SampleTime=ts_inv
  bemf_observer_ccaller : Subsystem  Commented=on
  bemf_observer_simulink : Subsystem
  bemf_observer_with_load_estimator_ccaller : Subsystem  Commented=on
  tag scope: motor_omega_hat_pu_dbv=global, motor_theta_hat_dbv=global
  wires:
  bemf_observer_simulink/1(omega_pu_hat) -> Unit Delay/1  "omega_hat_pu"
  bemf_observer_simulink/2(theta_hat) -> Unit Delay1/1  "theta_hat"
  ubeta_pu/1 -> bemf_observer_simulink/4(ubeta_pu)
  ualpha_pu/1 -> bemf_observer_simulink/3(ualpha_pu)
  ibeta_pu/1 -> bemf_observer_simulink/2(ibeta_pu)
  ialpha_pu/1 -> bemf_observer_simulink/1(ialpha_pu)
  Unit Delay/1 -> [motor_omega_hat_pu_dbv]
  Unit Delay1/1 -> [motor_theta_hat_dbv]

== system afe_rst_inv_psm_distributed_control_two_delays/INV-Modular/inv_leg_v/driver_board_v/motor_vector_control/current_ctrl ==
  iq_ref : Inport
  MTPA : Subsystem
      mask Display: disp('MTPA')
  dq_pi_with_vector_antiwindup : Subsystem
  id_ref : Subsystem
      settings: PortSchema="{\"entries\":[{\"content\":{\"sides\":[{\"content\":{},\"type\":\"ConnectorPlacement.EquallySpacedRectSide\",\"uuid\":\"42af5d69-f0eb-42c6-9e03-28c1d0757323\"},{\"content\":{\"connectorIds\":[\"Out1\"],\"side\":\"RIGHT\"},\"type\":\"ConnectorPlacement.EquallySpacedRectSide\",\"uuid\":\"dd68a9f9-d15f-4e57-9d9e-130889a7b90c\"},{\"content\":{\"connectorIds\":[\"In1\"],\"side\":\"TOP\"},\"type\":\"ConnectorPlacement.EquallySpacedRectSide\",\"uuid\":\"68c797a2-8439-4b8d-8368-b7485adf0676\"}]},\"type\":\"ConnectorPlacement.EquallySpacedConnector\",\"uuid\":\"693c5f1c-0580-4626-8f13-b27865dfb3ac\"}],\"packageUris\":[\"http://schema.mathworks.com/mf0/Connector/R2020b\"],\"version\":\"1.0\"}"
  idref/id : Scope  NumInputPorts=2
      settings: SampleTime=tc  ActiveDisplayYMinimum=-0.09748  ActiveDisplayYMaximum=0.07242
  iqref/iq : Scope  NumInputPorts=2
      settings: SampleTime=tc  ActiveDisplayYMinimum=-1.17759  ActiveDisplayYMaximum=0.13428  DataLoggingVariableName=ScopeData2
  ud : Outport
  uq : Outport  Port=2
  wires:
  [motor_iq_pu_dbv] -> MTPA/1(iq)  "iq"
  iq_ref/1 -> dq_pi_with_vector_antiwindup/3(iq_ref), iqref/iq/1  "iq"
  id_ref/1(id_ref) -> idref/id/1, dq_pi_with_vector_antiwindup/1(id_ref)
  dq_pi_with_vector_antiwindup/2(ctrl_q_u) -> uq/1
  dq_pi_with_vector_antiwindup/1(ctrl_d_u) -> ud/1
  MTPA/1(Id_ref_mtpa) -> id_ref/1(id_mtpa)  "id_ref"
  [motor_id_pu_dbv] -> dq_pi_with_vector_antiwindup/2(id), idref/id/2  "id"
  [motor_iq_pu_dbv] -> dq_pi_with_vector_antiwindup/4(iq), iqref/iq/2  "iq"

== system afe_rst_inv_psm_distributed_control_two_delays/INV-Modular/inv_leg_v/driver_board_v/motor_vector_control/current_transformation ==
  u : Inport
  v : Inport  Port=2
  w : Inport  Port=3
  gamma : Inport  Port=4
  alphabeta2dq : MATLAB Function  TreatAsAtomicUnit=on  SystemSampleTime=ts_inv
  uvw2alphabeta : MATLAB Function  TreatAsAtomicUnit=on  SystemSampleTime=ts_inv
  tag scope: motor_ialpha_pu_dbv=global, motor_ibeta_pu_dbv=global, motor_id_pu_dbv=global, motor_iq_pu_dbv=global
  wires:
  u/1 -> uvw2alphabeta/1(u)
  gamma/1 -> alphabeta2dq/3(gamma)
  uvw2alphabeta/1(alpha) -> alphabeta2dq/1(alpha), [motor_ialpha_pu_dbv]  "ialpha_pu"
  uvw2alphabeta/2(beta) -> alphabeta2dq/2(beta), [motor_ibeta_pu_dbv]  "ibeta_pu"
  v/1 -> uvw2alphabeta/2(v)
  alphabeta2dq/1(d) -> [motor_id_pu_dbv]  "id_pu"
  alphabeta2dq/2(q) -> [motor_iq_pu_dbv]  "iq_pu"
  w/1 -> uvw2alphabeta/3(w)

== system afe_rst_inv_psm_distributed_control_two_delays/INV-Modular/inv_leg_v/driver_board_v/voltage-current-acquisition/isu_measure ==
  is : Inport
  Gain : Gain  Gain=1/ibez
  Quantizer : Quantizer  QuantizationInterval=CurrentQuantization
  Unit Delay : UnitDelay  SampleTime=ts_afe
  Zero-Order Hold : ZeroOrderHold  SampleTime=ts_afe
  is_pu : Outport
  wires:
  Quantizer/1 -> Zero-Order Hold/1
  Gain/1 -> is_pu/1
  Zero-Order Hold/1 -> Unit Delay/1
  Unit Delay/1 -> Gain/1
  is/1 -> Quantizer/1

== system afe_rst_inv_psm_distributed_control_two_delays/INV-Modular/inv_leg_v/driver_board_v/voltage-current-acquisition/isv_fieldbus ==
  is : Inport
  Unit Delay : UnitDelay  SampleTime=ts_inv
  Unit Delay1 : UnitDelay  SampleTime=ts_inv
  Zero-Order Hold : ZeroOrderHold  SampleTime=ts_inv
  is_fb : Outport
  wires:
  Zero-Order Hold/1 -> Unit Delay/1
  is/1 -> Zero-Order Hold/1
  Unit Delay/1 -> Unit Delay1/1
  Unit Delay1/1 -> is_fb/1

== system afe_rst_inv_psm_distributed_control_two_delays/INV-Modular/inv_leg_v/driver_board_v/voltage-current-acquisition/isw_fieldbus ==
  is : Inport
  Unit Delay : UnitDelay  SampleTime=ts_inv
  Unit Delay1 : UnitDelay  SampleTime=ts_inv
  Zero-Order Hold : ZeroOrderHold  SampleTime=ts_inv
  is_fb : Outport
  wires:
  Zero-Order Hold/1 -> Unit Delay/1
  is/1 -> Zero-Order Hold/1
  Unit Delay/1 -> Unit Delay1/1
  Unit Delay1/1 -> is_fb/1

== system afe_rst_inv_psm_distributed_control_two_delays/INV-Modular/inv_leg_v/driver_board_v/voltage-current-acquisition/motor_phase_fieldbus ==
  motor_phase : Inport
  Unit Delay : UnitDelay  SampleTime=ts_inv
  Unit Delay1 : UnitDelay  SampleTime=ts_inv
  Zero-Order Hold : ZeroOrderHold  SampleTime=ts_inv
  motor_phase_fb : Outport
  wires:
  Zero-Order Hold/1 -> Unit Delay/1
  motor_phase/1 -> Zero-Order Hold/1
  Unit Delay/1 -> Unit Delay1/1
  Unit Delay1/1 -> motor_phase_fb/1

== system afe_rst_inv_psm_distributed_control_two_delays/INV-Modular/inv_leg_v/driver_board_v/voltage-current-acquisition/motor_torque_fieldbus ==
  us : Inport
  Unit Delay : UnitDelay  SampleTime=ts_inv
  Unit Delay1 : UnitDelay  SampleTime=ts_inv
  Zero-Order Hold : ZeroOrderHold  SampleTime=ts_inv
  us_fb : Outport
  wires:
  Zero-Order Hold/1 -> Unit Delay/1
  us/1 -> Zero-Order Hold/1
  Unit Delay/1 -> Unit Delay1/1
  Unit Delay1/1 -> us_fb/1

== system afe_rst_inv_psm_distributed_control_two_delays/INV-Modular/inv_leg_v/driver_board_v/voltage-current-acquisition/usu_ctrl_fieldbus ==
  u_ctrl : Inport
  Unit Delay : UnitDelay  SampleTime=ts_inv
  Unit Delay1 : UnitDelay  SampleTime=ts_inv
  Zero-Order Hold : ZeroOrderHold  SampleTime=ts_inv
  u_ctrl_fb : Outport
  wires:
  Zero-Order Hold/1 -> Unit Delay/1
  u_ctrl/1 -> Zero-Order Hold/1
  Unit Delay/1 -> Unit Delay1/1
  Unit Delay1/1 -> u_ctrl_fb/1

== system afe_rst_inv_psm_distributed_control_two_delays/INV-Modular/inv_leg_v/driver_board_v/voltage-current-acquisition/usu_fieldbus ==
  us : Inport
  Unit Delay : UnitDelay  SampleTime=ts_inv
  Unit Delay1 : UnitDelay  SampleTime=ts_inv
  Zero-Order Hold : ZeroOrderHold  SampleTime=ts_inv
  us_fb : Outport
  wires:
  Zero-Order Hold/1 -> Unit Delay/1
  us/1 -> Zero-Order Hold/1
  Unit Delay/1 -> Unit Delay1/1
  Unit Delay1/1 -> us_fb/1

== system afe_rst_inv_psm_distributed_control_two_delays/INV-Modular/inv_leg_v/driver_board_v/voltage-current-acquisition/usv_measure ==
  us : Inport
  Gain : Gain  Gain=1/ubez
  Quantizer : Quantizer  QuantizationInterval=CurrentQuantization
  Unit Delay : UnitDelay  SampleTime=ts_inv
  Zero-Order Hold : ZeroOrderHold  SampleTime=ts_inv
  us_pu : Outport
  wires:
  us/1 -> Quantizer/1
  Unit Delay/1 -> Gain/1
  Zero-Order Hold/1 -> Unit Delay/1
  Gain/1 -> us_pu/1
  Quantizer/1 -> Zero-Order Hold/1

== system afe_rst_inv_psm_distributed_control_two_delays/INV-Modular/inv_leg_v/driver_board_v/voltage-current-acquisition/usw_ctrl_fieldbus ==
  u_ctrl : Inport
  Unit Delay : UnitDelay  SampleTime=ts_inv
  Unit Delay1 : UnitDelay  SampleTime=ts_inv
  Zero-Order Hold : ZeroOrderHold  SampleTime=ts_inv
  u_ctrl_fb : Outport
  wires:
  Zero-Order Hold/1 -> Unit Delay/1
  u_ctrl/1 -> Zero-Order Hold/1
  Unit Delay/1 -> Unit Delay1/1
  Unit Delay1/1 -> u_ctrl_fb/1

== system afe_rst_inv_psm_distributed_control_two_delays/INV-Modular/inv_leg_v/driver_board_v/voltage-current-acquisition/usw_fieldbus ==
  us : Inport
  Unit Delay : UnitDelay  SampleTime=ts_inv
  Unit Delay1 : UnitDelay  SampleTime=ts_inv
  Zero-Order Hold : ZeroOrderHold  SampleTime=ts_inv
  us_fb : Outport
  wires:
  Zero-Order Hold/1 -> Unit Delay/1
  us/1 -> Zero-Order Hold/1
  Unit Delay/1 -> Unit Delay1/1
  Unit Delay1/1 -> us_fb/1

== system afe_rst_inv_psm_distributed_control_two_delays/INV-Modular/inv_leg_v/modulator/sv_pwm/modulator ==
  mv : Inport
  Bus Creator : BusCreator  Inputs=2
  PWM generator : Subsystem  mask{f=fPWM_INV, ph=0, m_up=0.98, m_low=0.02, dead_time=dead_time_INV, vg_firing=15, polarity=1}
      mask prompts: f "Frequency"; ph "Phase"; m_up "Max Input Modulation Value"; m_low "Min Input Modulation Value"; dead_time "Dead Time"; vg_firing "Gate Voltage"
  firing_gates : Outport
  wires:
  mv/1 -> PWM generator/1(m_index)
  PWM generator/2(m2) -> Bus Creator/2  "pwm_v_bottom"
  Bus Creator/1 -> firing_gates/1
  PWM generator/1(m1) -> Bus Creator/1  "pwm_v_top"

== system afe_rst_inv_psm_distributed_control_two_delays/INV-Modular/inv_leg_w/driver_board_w/motor_vector_control/bemf_observer ==
  ialpha_pu : Inport
  ibeta_pu : Inport  Port=2
  ualpha_pu : Inport  Port=3
  ubeta_pu : Inport  Port=4
  Unit Delay : UnitDelay  SampleTime=ts_inv
  Unit Delay1 : UnitDelay  SampleTime=ts_inv
  bemf_observer_ccaller : Subsystem  Commented=on
  bemf_observer_simulink : Subsystem
  bemf_observer_with_load_estimator_ccaller : Subsystem  Commented=on
  tag scope: motor_omega_hat_pu_dbw=global, motor_theta_hat_dbw=global
  wires:
  bemf_observer_simulink/1(omega_pu_hat) -> Unit Delay/1  "omega_hat_pu"
  ubeta_pu/1 -> bemf_observer_simulink/4(ubeta_pu)
  ualpha_pu/1 -> bemf_observer_simulink/3(ualpha_pu)
  ibeta_pu/1 -> bemf_observer_simulink/2(ibeta_pu)
  ialpha_pu/1 -> bemf_observer_simulink/1(ialpha_pu)
  Unit Delay/1 -> [motor_omega_hat_pu_dbw]
  Unit Delay1/1 -> [motor_theta_hat_dbw]
  bemf_observer_simulink/2(theta_hat) -> Unit Delay1/1  "theta_hat"

== system afe_rst_inv_psm_distributed_control_two_delays/INV-Modular/inv_leg_w/driver_board_w/motor_vector_control/current_ctrl ==
  iq_ref : Inport
  MTPA : Subsystem
      mask Display: disp('MTPA')
  dq_pi_with_vector_antiwindup : Subsystem
  id_ref : Subsystem
      settings: PortSchema="{\"entries\":[{\"content\":{\"sides\":[{\"content\":{},\"type\":\"ConnectorPlacement.EquallySpacedRectSide\",\"uuid\":\"42af5d69-f0eb-42c6-9e03-28c1d0757323\"},{\"content\":{\"connectorIds\":[\"Out1\"],\"side\":\"RIGHT\"},\"type\":\"ConnectorPlacement.EquallySpacedRectSide\",\"uuid\":\"dd68a9f9-d15f-4e57-9d9e-130889a7b90c\"},{\"content\":{\"connectorIds\":[\"In1\"],\"side\":\"TOP\"},\"type\":\"ConnectorPlacement.EquallySpacedRectSide\",\"uuid\":\"68c797a2-8439-4b8d-8368-b7485adf0676\"}]},\"type\":\"ConnectorPlacement.EquallySpacedConnector\",\"uuid\":\"693c5f1c-0580-4626-8f13-b27865dfb3ac\"}],\"packageUris\":[\"http://schema.mathworks.com/mf0/Connector/R2020b\"],\"version\":\"1.0\"}"
  idref/id : Scope  NumInputPorts=2
      settings: SampleTime=tc  ActiveDisplayYMinimum=-0.25498  ActiveDisplayYMaximum=0.16065
  iqref/iq : Scope  NumInputPorts=2
      settings: SampleTime=tc  ActiveDisplayYMinimum=-0.66775  ActiveDisplayYMaximum=0.07588  DataLoggingVariableName=ScopeData2
  ud : Outport
  uq : Outport  Port=2
  wires:
  [motor_iq_pu_dbw] -> MTPA/1(iq)  "iq"
  iq_ref/1 -> iqref/iq/1, dq_pi_with_vector_antiwindup/3(iq_ref)  "iq"
  id_ref/1(id_ref) -> idref/id/1, dq_pi_with_vector_antiwindup/1(id_ref)
  dq_pi_with_vector_antiwindup/2(ctrl_q_u) -> uq/1
  dq_pi_with_vector_antiwindup/1(ctrl_d_u) -> ud/1
  MTPA/1(Id_ref_mtpa) -> id_ref/1(id_mtpa)  "id_ref"
  [motor_id_pu_dbw] -> idref/id/2, dq_pi_with_vector_antiwindup/2(id)  "id"
  [motor_iq_pu_dbw] -> iqref/iq/2, dq_pi_with_vector_antiwindup/4(iq)  "iq"

== system afe_rst_inv_psm_distributed_control_two_delays/INV-Modular/inv_leg_w/driver_board_w/motor_vector_control/current_transformation ==
  u : Inport
  v : Inport  Port=2
  w : Inport  Port=3
  gamma : Inport  Port=4
  alphabeta2dq : MATLAB Function  TreatAsAtomicUnit=on  SystemSampleTime=ts_inv
  uvw2alphabeta : MATLAB Function  TreatAsAtomicUnit=on  SystemSampleTime=ts_inv
  tag scope: motor_ialpha_pu_dbw=global, motor_ibeta_pu_dbw=global, motor_id_pu_dbw=global, motor_iq_pu_dbw=global
  wires:
  u/1 -> uvw2alphabeta/1(u)
  uvw2alphabeta/1(alpha) -> alphabeta2dq/1(alpha), [motor_ialpha_pu_dbw]  "ialpha_pu"
  uvw2alphabeta/2(beta) -> alphabeta2dq/2(beta), [motor_ibeta_pu_dbw]  "ibeta_pu"
  v/1 -> uvw2alphabeta/2(v)
  alphabeta2dq/1(d) -> [motor_id_pu_dbw]  "id_pu"
  alphabeta2dq/2(q) -> [motor_iq_pu_dbw]  "iq_pu"
  w/1 -> uvw2alphabeta/3(w)
  gamma/1 -> alphabeta2dq/3(gamma)

== system afe_rst_inv_psm_distributed_control_two_delays/INV-Modular/inv_leg_w/driver_board_w/voltage-current-acquisition/isu_fieldbus ==
  is : Inport
  Unit Delay : UnitDelay  SampleTime=ts_inv
  Unit Delay1 : UnitDelay  SampleTime=ts_inv
  Zero-Order Hold : ZeroOrderHold  SampleTime=ts_inv
  is_fb : Outport
  wires:
  Zero-Order Hold/1 -> Unit Delay/1
  is/1 -> Zero-Order Hold/1
  Unit Delay/1 -> Unit Delay1/1
  Unit Delay1/1 -> is_fb/1

== system afe_rst_inv_psm_distributed_control_two_delays/INV-Modular/inv_leg_w/driver_board_w/voltage-current-acquisition/isv_fieldbus ==
  is : Inport
  Unit Delay : UnitDelay  SampleTime=ts_inv
  Unit Delay1 : UnitDelay  SampleTime=ts_inv
  Zero-Order Hold : ZeroOrderHold  SampleTime=ts_inv
  is_fb : Outport
  wires:
  Zero-Order Hold/1 -> Unit Delay/1
  is/1 -> Zero-Order Hold/1
  Unit Delay/1 -> Unit Delay1/1
  Unit Delay1/1 -> is_fb/1

== system afe_rst_inv_psm_distributed_control_two_delays/INV-Modular/inv_leg_w/driver_board_w/voltage-current-acquisition/isw_measure_and_normalization ==
  is : Inport
  Gain : Gain  Gain=1/ibez
  Quantizer : Quantizer  QuantizationInterval=CurrentQuantization
  Unit Delay : UnitDelay  SampleTime=ts_afe
  Zero-Order Hold : ZeroOrderHold  SampleTime=ts_afe
  is_pu : Outport
  wires:
  is/1 -> Quantizer/1
  Unit Delay/1 -> Gain/1
  Zero-Order Hold/1 -> Unit Delay/1
  Gain/1 -> is_pu/1
  Quantizer/1 -> Zero-Order Hold/1

== system afe_rst_inv_psm_distributed_control_two_delays/INV-Modular/inv_leg_w/driver_board_w/voltage-current-acquisition/motor_phase_fieldbus ==
  motor_phase : Inport
  Unit Delay : UnitDelay  SampleTime=ts_inv
  Unit Delay1 : UnitDelay  SampleTime=ts_inv
  Zero-Order Hold : ZeroOrderHold  SampleTime=ts_inv
  motor_phase_fb : Outport
  wires:
  Zero-Order Hold/1 -> Unit Delay/1
  motor_phase/1 -> Zero-Order Hold/1
  Unit Delay/1 -> Unit Delay1/1
  Unit Delay1/1 -> motor_phase_fb/1

== system afe_rst_inv_psm_distributed_control_two_delays/INV-Modular/inv_leg_w/driver_board_w/voltage-current-acquisition/motor_torque_fieldbus ==
  motor_torque_ref : Inport
  Unit Delay : UnitDelay  SampleTime=ts_inv
  Unit Delay1 : UnitDelay  SampleTime=ts_inv
  Zero-Order Hold : ZeroOrderHold  SampleTime=ts_inv
  motor_torque_ref_fb : Outport
  wires:
  Zero-Order Hold/1 -> Unit Delay/1
  motor_torque_ref/1 -> Zero-Order Hold/1
  Unit Delay/1 -> Unit Delay1/1
  Unit Delay1/1 -> motor_torque_ref_fb/1

== system afe_rst_inv_psm_distributed_control_two_delays/INV-Modular/inv_leg_w/driver_board_w/voltage-current-acquisition/usu_ctrl_fieldbus ==
  u_ctrl : Inport
  Unit Delay : UnitDelay  SampleTime=ts_inv
  Unit Delay1 : UnitDelay  SampleTime=ts_inv
  Zero-Order Hold : ZeroOrderHold  SampleTime=ts_inv
  u_ctrl_fb : Outport
  wires:
  Zero-Order Hold/1 -> Unit Delay/1
  u_ctrl/1 -> Zero-Order Hold/1
  Unit Delay/1 -> Unit Delay1/1
  Unit Delay1/1 -> u_ctrl_fb/1
